simulink model "DWPT_250k_60V_1200W"  (R2026b)
settings: Solver=ode3  StopTime=0.03  FixedStep=Ts  MaxStep=1.0E-7  RelTol=1e-4  AbsTol=1e-6
model workspace (MAT data in the model file):
  CP1 = 8.25994623514e-08
  CS = 4.09933827549e-08
  CT1 = 8.13830913262e-08
  Cout = 0.0022
  Goff = 1e-08
  Ki = 20
  Kp = 0.015
  LP1 = 9.88658918421e-06
  LS = 9.88658918421e-06
  LT1 = 4.97996239716e-06
  M1 = 6.87234810809e-06
  Mdesign = 6.87234810809e-06
  RL = 3
  RP1 = 0.0171021142042
  RS = 0.0171021142042
  RT1 = 0.01
  RonSR = 0.003
  RonTx = 0.003
  Ts = 1e-08
  Vavailable = 69
  Vdc = 50
  Vtarget = 60
  averageCycles = 1250
  bodyRon = 0.01
  bodyVf = 0.8
  closedLoop = 1
  deadTime = 4e-08
  f = 250000
  initialOutputVoltage = 0
  k = 0.695118203056
  samplesPerPeriod = 400
  softStart = 0.02
  srDeadTime = 4e-08
  srEnabled = 1
  srThreshold = 0.25
  voltageHeadroom = 1.15
undefined symbols (not defined in the file or in its folder): ee_sli_rtmsupport, G, gcbh
libraries: sl_signal_attributes x63, eeGeneralControl x37, fl_lib x32, nesl_utility x28, eeGeneralMeasurement x14, ee_lib x8, dspfdesign x1
(part 3 of 3)

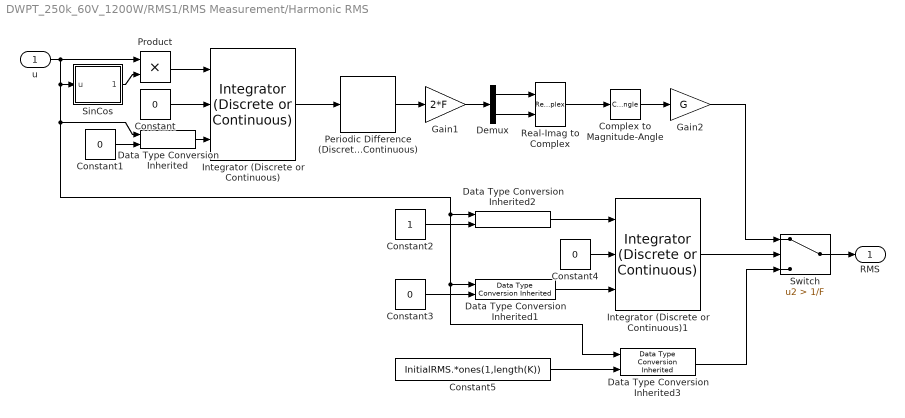
== system DWPT_250k_60V_1200W/RMS1/RMS Measurement/Harmonic RMS ==
  u : Inport
  Complex to Magnitude-Angle : ComplexToMagnitudeAngle  Output=Magnitude
  Constant{,1,3..4} (4 alike) : Constant  Value=0
  Constant2 : Constant
  Constant5 : Constant  Value=InitialRMS.*ones(1,length(K))
  Data Type Conversion Inherited{,1..3} (4 alike) : sl_signal_attributes/Data Type Conversion Inherited  ConvertRealWorld=Real World Value  DoSatur=off
  Demux : Demux  Outputs=2
  Gain1 : Gain  Gain=2*F
  Gain2 : Gain  Gain=G
  Integrator (Discrete or Continuous) : eeGeneralControl/Integrator (Discrete or Continuous)  LabelModeActiveChoice=Continuous  IntegratorMethod=Integration: Forward Euler  ExternalReset=level  LimitType=Anti-windup  B=inf  A=-inf  Ts=Ts
  Integrator (Discrete or Continuous)1 : eeGeneralControl/Integrator (Discrete or Continuous)  LabelModeActiveChoice=Continuous  IntegratorMethod=Integration: Forward Euler  ExternalReset=level  LimitType=Anti-windup  B=2/F  A=-inf  Ts=Ts
  Periodic Difference (Discrete or Continuous) : eeGeneralMeasurement/Periodic Difference (Discrete or Continuous)  LabelModeActiveChoice=Continuous  F=F  Ts=Ts
      link override Continuous/Transport Delay: BufferSize=2^nextpow2(samplesPerPeriod*averageCycles+1024)
  Product : Product
  Real-Imag to Complex : RealImagToComplex
  SinCos : Subsystem
  Switch : Switch  Criteria=u2 > Threshold  Threshold=1/F  SaturateOnIntegerOverflow=off  InputSameDT=off
  RMS : Outport  VectorParamsAs1DForOutWhenUnconnected=off
  wires:
  Switch/1 -> RMS/1
  Gain2/1 -> Switch/1
  Constant2/1 -> Data Type Conversion Inherited2/2
  Constant3/1 -> Data Type Conversion Inherited1/2
  Constant4/1 -> Integrator (Discrete or Continuous)1/2
  Data Type Conversion Inherited3/1 -> Switch/3
  Constant5/1 -> Data Type Conversion Inherited3/2
  Data Type Conversion Inherited2/1 -> Integrator (Discrete or Continuous)1/1
  Data Type Conversion Inherited1/1 -> Integrator (Discrete or Continuous)1/3
  Integrator (Discrete or Continuous)1/1 -> Switch/2
  Constant1/1 -> Data Type Conversion Inherited/2
  Data Type Conversion Inherited/1 -> Integrator (Discrete or Continuous)/3
  Integrator (Discrete or Continuous)/1 -> Periodic Difference (Discrete or Continuous)/1
  Constant/1 -> Integrator (Discrete or Continuous)/2
  Demux/2 -> Real-Imag to Complex/2
  u/1 -> SinCos/1(u), Data Type Conversion Inherited/1, Data Type Conversion Inherited2/1, Data Type Conversion Inherited1/1, Data Type Conversion Inherited3/1, Product/1
  Periodic Difference (Discrete or Continuous)/1 -> Gain1/1
  Real-Imag to Complex/1 -> Complex to Magnitude-Angle/1
  Demux/1 -> Real-Imag to Complex/1
  SinCos/1(SinCos) -> Product/2
  Gain1/1 -> Demux/1
  Product/1 -> Integrator (Discrete or Continuous)/1
  Complex to Magnitude-Angle/1 -> Gain2/1

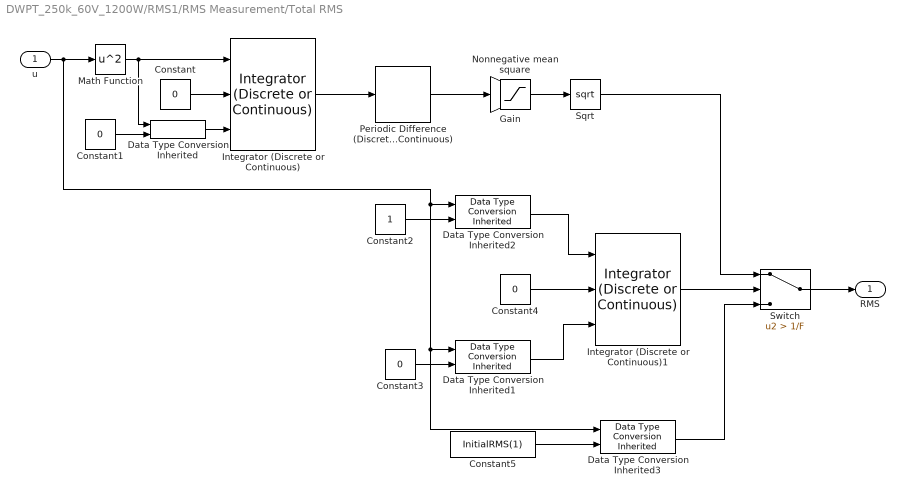
== system DWPT_250k_60V_1200W/RMS1/RMS Measurement/Total RMS ==
  u : Inport
  Constant{,1,3..4} (4 alike) : Constant  Value=0
  Constant2 : Constant
  Constant5 : Constant  Value=InitialRMS(1)
  Data Type Conversion Inherited{,1..3} (4 alike) : sl_signal_attributes/Data Type Conversion Inherited  ConvertRealWorld=Real World Value  DoSatur=off
  Gain : Gain  Gain=F
  Integrator (Discrete or Continuous) : eeGeneralControl/Integrator (Discrete or Continuous)  LabelModeActiveChoice=Continuous  IntegratorMethod=Integration: Forward Euler  ExternalReset=level  LimitType=Anti-windup  B=inf  A=-inf  Ts=Ts
  Integrator (Discrete or Continuous)1 : eeGeneralControl/Integrator (Discrete or Continuous)  LabelModeActiveChoice=Continuous  IntegratorMethod=Integration: Forward Euler  ExternalReset=level  LimitType=Anti-windup  B=2/F  A=-inf  Ts=Ts
  Math Function : Math  Operator=square  SignedPower=on
  Nonnegative mean square : Saturate  UpperLimit=inf  LowerLimit=0
  Periodic Difference (Discrete or Continuous) : eeGeneralMeasurement/Periodic Difference (Discrete or Continuous)  LabelModeActiveChoice=Continuous  F=F  Ts=Ts
      link override Continuous/Transport Delay: BufferSize=2^nextpow2(samplesPerPeriod*averageCycles+1024)
  Sqrt : Sqrt
  Switch : Switch  Criteria=u2 > Threshold  Threshold=1/F  SaturateOnIntegerOverflow=off  InputSameDT=off
  RMS : Outport  VectorParamsAs1DForOutWhenUnconnected=off
  wires:
  Sqrt/1 -> Switch/1
  Switch/1 -> RMS/1
  Constant2/1 -> Data Type Conversion Inherited2/2
  Constant3/1 -> Data Type Conversion Inherited1/2
  Constant4/1 -> Integrator (Discrete or Continuous)1/2
  Data Type Conversion Inherited3/1 -> Switch/3
  Constant5/1 -> Data Type Conversion Inherited3/2
  Data Type Conversion Inherited2/1 -> Integrator (Discrete or Continuous)1/1
  Data Type Conversion Inherited1/1 -> Integrator (Discrete or Continuous)1/3
  Integrator (Discrete or Continuous)1/1 -> Switch/2
  Constant1/1 -> Data Type Conversion Inherited/2
  Data Type Conversion Inherited/1 -> Integrator (Discrete or Continuous)/3
  Periodic Difference (Discrete or Continuous)/1 -> Gain/1
  Integrator (Discrete or Continuous)/1 -> Periodic Difference (Discrete or Continuous)/1
  u/1 -> Math Function/1, Data Type Conversion Inherited2/1, Data Type Conversion Inherited3/1, Data Type Conversion Inherited1/1
  Math Function/1 -> Integrator (Discrete or Continuous)/1, Data Type Conversion Inherited/1
  Constant/1 -> Integrator (Discrete or Continuous)/2
  Gain/1 -> Nonnegative mean square/1
  Nonnegative mean square/1 -> Sqrt/1

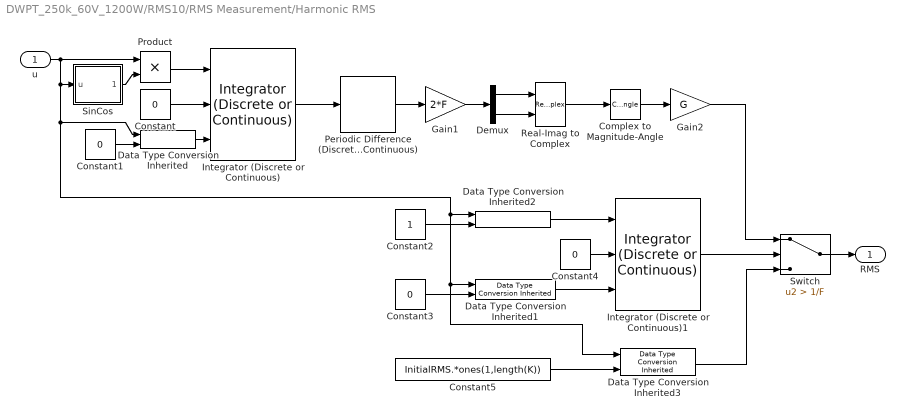
== system DWPT_250k_60V_1200W/RMS10/RMS Measurement/Harmonic RMS ==
  u : Inport
  Complex to Magnitude-Angle : ComplexToMagnitudeAngle  Output=Magnitude
  Constant{,1,3..4} (4 alike) : Constant  Value=0
  Constant2 : Constant
  Constant5 : Constant  Value=InitialRMS.*ones(1,length(K))
  Data Type Conversion Inherited{,1..3} (4 alike) : sl_signal_attributes/Data Type Conversion Inherited  ConvertRealWorld=Real World Value  DoSatur=off
  Demux : Demux  Outputs=2
  Gain1 : Gain  Gain=2*F
  Gain2 : Gain  Gain=G
  Integrator (Discrete or Continuous) : eeGeneralControl/Integrator (Discrete or Continuous)  LabelModeActiveChoice=Continuous  IntegratorMethod=Integration: Forward Euler  ExternalReset=level  LimitType=Anti-windup  B=inf  A=-inf  Ts=Ts
  Integrator (Discrete or Continuous)1 : eeGeneralControl/Integrator (Discrete or Continuous)  LabelModeActiveChoice=Continuous  IntegratorMethod=Integration: Forward Euler  ExternalReset=level  LimitType=Anti-windup  B=2/F  A=-inf  Ts=Ts
  Periodic Difference (Discrete or Continuous) : eeGeneralMeasurement/Periodic Difference (Discrete or Continuous)  LabelModeActiveChoice=Continuous  F=F  Ts=Ts
      link override Continuous/Transport Delay: BufferSize=2^nextpow2(samplesPerPeriod*averageCycles+1024)
  Product : Product
  Real-Imag to Complex : RealImagToComplex
  SinCos : Subsystem
  Switch : Switch  Criteria=u2 > Threshold  Threshold=1/F  SaturateOnIntegerOverflow=off  InputSameDT=off
  RMS : Outport  VectorParamsAs1DForOutWhenUnconnected=off
  wires:
  Switch/1 -> RMS/1
  Gain2/1 -> Switch/1
  Constant2/1 -> Data Type Conversion Inherited2/2
  Constant3/1 -> Data Type Conversion Inherited1/2
  Constant4/1 -> Integrator (Discrete or Continuous)1/2
  Data Type Conversion Inherited3/1 -> Switch/3
  Constant5/1 -> Data Type Conversion Inherited3/2
  Data Type Conversion Inherited2/1 -> Integrator (Discrete or Continuous)1/1
  Data Type Conversion Inherited1/1 -> Integrator (Discrete or Continuous)1/3
  Integrator (Discrete or Continuous)1/1 -> Switch/2
  Constant1/1 -> Data Type Conversion Inherited/2
  Data Type Conversion Inherited/1 -> Integrator (Discrete or Continuous)/3
  Integrator (Discrete or Continuous)/1 -> Periodic Difference (Discrete or Continuous)/1
  Constant/1 -> Integrator (Discrete or Continuous)/2
  Demux/2 -> Real-Imag to Complex/2
  u/1 -> SinCos/1(u), Data Type Conversion Inherited/1, Data Type Conversion Inherited2/1, Data Type Conversion Inherited1/1, Data Type Conversion Inherited3/1, Product/1
  Periodic Difference (Discrete or Continuous)/1 -> Gain1/1
  Real-Imag to Complex/1 -> Complex to Magnitude-Angle/1
  Demux/1 -> Real-Imag to Complex/1
  SinCos/1(SinCos) -> Product/2
  Gain1/1 -> Demux/1
  Product/1 -> Integrator (Discrete or Continuous)/1
  Complex to Magnitude-Angle/1 -> Gain2/1

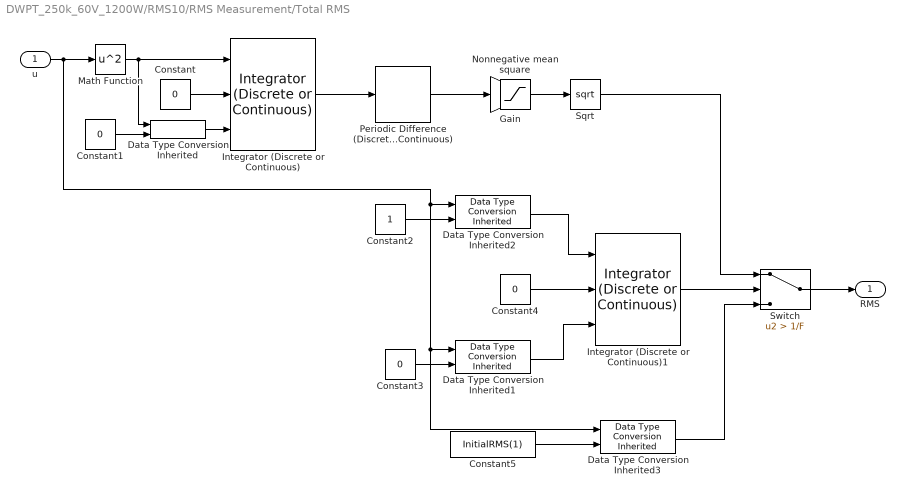
== system DWPT_250k_60V_1200W/RMS10/RMS Measurement/Total RMS ==
  u : Inport
  Constant{,1,3..4} (4 alike) : Constant  Value=0
  Constant2 : Constant
  Constant5 : Constant  Value=InitialRMS(1)
  Data Type Conversion Inherited{,1..3} (4 alike) : sl_signal_attributes/Data Type Conversion Inherited  ConvertRealWorld=Real World Value  DoSatur=off
  Gain : Gain  Gain=F
  Integrator (Discrete or Continuous) : eeGeneralControl/Integrator (Discrete or Continuous)  LabelModeActiveChoice=Continuous  IntegratorMethod=Integration: Forward Euler  ExternalReset=level  LimitType=Anti-windup  B=inf  A=-inf  Ts=Ts
  Integrator (Discrete or Continuous)1 : eeGeneralControl/Integrator (Discrete or Continuous)  LabelModeActiveChoice=Continuous  IntegratorMethod=Integration: Forward Euler  ExternalReset=level  LimitType=Anti-windup  B=2/F  A=-inf  Ts=Ts
  Math Function : Math  Operator=square  SignedPower=on
  Nonnegative mean square : Saturate  UpperLimit=inf  LowerLimit=0
  Periodic Difference (Discrete or Continuous) : eeGeneralMeasurement/Periodic Difference (Discrete or Continuous)  LabelModeActiveChoice=Continuous  F=F  Ts=Ts
      link override Continuous/Transport Delay: BufferSize=2^nextpow2(samplesPerPeriod*averageCycles+1024)
  Sqrt : Sqrt
  Switch : Switch  Criteria=u2 > Threshold  Threshold=1/F  SaturateOnIntegerOverflow=off  InputSameDT=off
  RMS : Outport  VectorParamsAs1DForOutWhenUnconnected=off
  wires:
  Sqrt/1 -> Switch/1
  Switch/1 -> RMS/1
  Constant2/1 -> Data Type Conversion Inherited2/2
  Constant3/1 -> Data Type Conversion Inherited1/2
  Constant4/1 -> Integrator (Discrete or Continuous)1/2
  Data Type Conversion Inherited3/1 -> Switch/3
  Constant5/1 -> Data Type Conversion Inherited3/2
  Data Type Conversion Inherited2/1 -> Integrator (Discrete or Continuous)1/1
  Data Type Conversion Inherited1/1 -> Integrator (Discrete or Continuous)1/3
  Integrator (Discrete or Continuous)1/1 -> Switch/2
  Constant1/1 -> Data Type Conversion Inherited/2
  Data Type Conversion Inherited/1 -> Integrator (Discrete or Continuous)/3
  Periodic Difference (Discrete or Continuous)/1 -> Gain/1
  Integrator (Discrete or Continuous)/1 -> Periodic Difference (Discrete or Continuous)/1
  u/1 -> Math Function/1, Data Type Conversion Inherited2/1, Data Type Conversion Inherited3/1, Data Type Conversion Inherited1/1
  Math Function/1 -> Integrator (Discrete or Continuous)/1, Data Type Conversion Inherited/1
  Constant/1 -> Integrator (Discrete or Continuous)/2
  Gain/1 -> Nonnegative mean square/1
  Nonnegative mean square/1 -> Sqrt/1

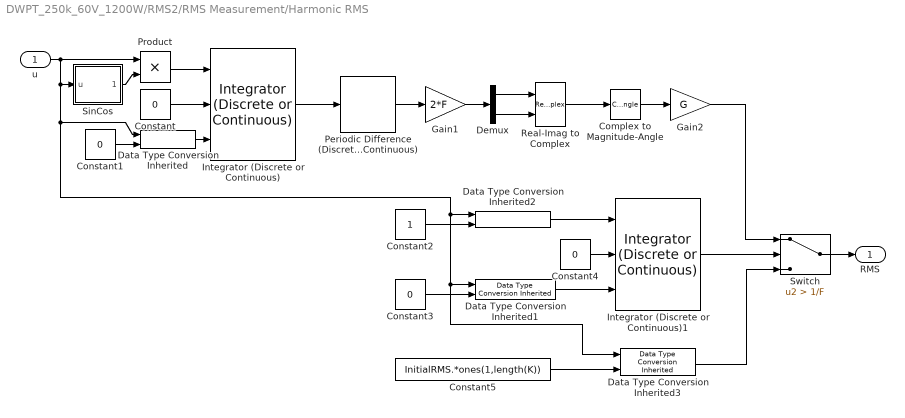
== system DWPT_250k_60V_1200W/RMS2/RMS Measurement/Harmonic RMS ==
  u : Inport
  Complex to Magnitude-Angle : ComplexToMagnitudeAngle  Output=Magnitude
  Constant{,1,3..4} (4 alike) : Constant  Value=0
  Constant2 : Constant
  Constant5 : Constant  Value=InitialRMS.*ones(1,length(K))
  Data Type Conversion Inherited{,1..3} (4 alike) : sl_signal_attributes/Data Type Conversion Inherited  ConvertRealWorld=Real World Value  DoSatur=off
  Demux : Demux  Outputs=2
  Gain1 : Gain  Gain=2*F
  Gain2 : Gain  Gain=G
  Integrator (Discrete or Continuous) : eeGeneralControl/Integrator (Discrete or Continuous)  LabelModeActiveChoice=Continuous  IntegratorMethod=Integration: Forward Euler  ExternalReset=level  LimitType=Anti-windup  B=inf  A=-inf  Ts=Ts
  Integrator (Discrete or Continuous)1 : eeGeneralControl/Integrator (Discrete or Continuous)  LabelModeActiveChoice=Continuous  IntegratorMethod=Integration: Forward Euler  ExternalReset=level  LimitType=Anti-windup  B=2/F  A=-inf  Ts=Ts
  Periodic Difference (Discrete or Continuous) : eeGeneralMeasurement/Periodic Difference (Discrete or Continuous)  LabelModeActiveChoice=Continuous  F=F  Ts=Ts
      link override Continuous/Transport Delay: BufferSize=2^nextpow2(samplesPerPeriod*averageCycles+1024)
  Product : Product
  Real-Imag to Complex : RealImagToComplex
  SinCos : Subsystem
  Switch : Switch  Criteria=u2 > Threshold  Threshold=1/F  SaturateOnIntegerOverflow=off  InputSameDT=off
  RMS : Outport  VectorParamsAs1DForOutWhenUnconnected=off
  wires:
  Switch/1 -> RMS/1
  Gain2/1 -> Switch/1
  Constant2/1 -> Data Type Conversion Inherited2/2
  Constant3/1 -> Data Type Conversion Inherited1/2
  Constant4/1 -> Integrator (Discrete or Continuous)1/2
  Data Type Conversion Inherited3/1 -> Switch/3
  Constant5/1 -> Data Type Conversion Inherited3/2
  Data Type Conversion Inherited2/1 -> Integrator (Discrete or Continuous)1/1
  Data Type Conversion Inherited1/1 -> Integrator (Discrete or Continuous)1/3
  Integrator (Discrete or Continuous)1/1 -> Switch/2
  Constant1/1 -> Data Type Conversion Inherited/2
  Data Type Conversion Inherited/1 -> Integrator (Discrete or Continuous)/3
  Integrator (Discrete or Continuous)/1 -> Periodic Difference (Discrete or Continuous)/1
  Constant/1 -> Integrator (Discrete or Continuous)/2
  Demux/2 -> Real-Imag to Complex/2
  u/1 -> SinCos/1(u), Data Type Conversion Inherited/1, Data Type Conversion Inherited2/1, Data Type Conversion Inherited1/1, Data Type Conversion Inherited3/1, Product/1
  Periodic Difference (Discrete or Continuous)/1 -> Gain1/1
  Real-Imag to Complex/1 -> Complex to Magnitude-Angle/1
  Demux/1 -> Real-Imag to Complex/1
  SinCos/1(SinCos) -> Product/2
  Gain1/1 -> Demux/1
  Product/1 -> Integrator (Discrete or Continuous)/1
  Complex to Magnitude-Angle/1 -> Gain2/1

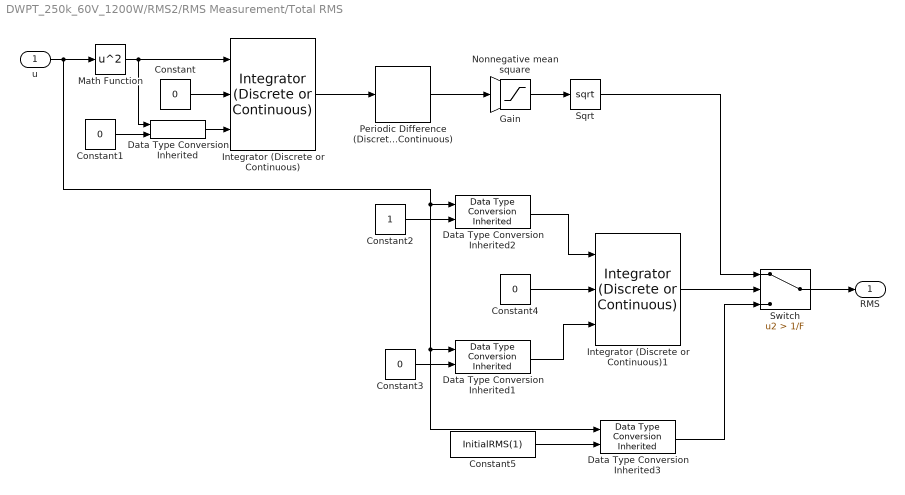
== system DWPT_250k_60V_1200W/RMS2/RMS Measurement/Total RMS ==
  u : Inport
  Constant{,1,3..4} (4 alike) : Constant  Value=0
  Constant2 : Constant
  Constant5 : Constant  Value=InitialRMS(1)
  Data Type Conversion Inherited{,1..3} (4 alike) : sl_signal_attributes/Data Type Conversion Inherited  ConvertRealWorld=Real World Value  DoSatur=off
  Gain : Gain  Gain=F
  Integrator (Discrete or Continuous) : eeGeneralControl/Integrator (Discrete or Continuous)  LabelModeActiveChoice=Continuous  IntegratorMethod=Integration: Forward Euler  ExternalReset=level  LimitType=Anti-windup  B=inf  A=-inf  Ts=Ts
  Integrator (Discrete or Continuous)1 : eeGeneralControl/Integrator (Discrete or Continuous)  LabelModeActiveChoice=Continuous  IntegratorMethod=Integration: Forward Euler  ExternalReset=level  LimitType=Anti-windup  B=2/F  A=-inf  Ts=Ts
  Math Function : Math  Operator=square  SignedPower=on
  Nonnegative mean square : Saturate  UpperLimit=inf  LowerLimit=0
  Periodic Difference (Discrete or Continuous) : eeGeneralMeasurement/Periodic Difference (Discrete or Continuous)  LabelModeActiveChoice=Continuous  F=F  Ts=Ts
      link override Continuous/Transport Delay: BufferSize=2^nextpow2(samplesPerPeriod*averageCycles+1024)
  Sqrt : Sqrt
  Switch : Switch  Criteria=u2 > Threshold  Threshold=1/F  SaturateOnIntegerOverflow=off  InputSameDT=off
  RMS : Outport  VectorParamsAs1DForOutWhenUnconnected=off
  wires:
  Sqrt/1 -> Switch/1
  Switch/1 -> RMS/1
  Constant2/1 -> Data Type Conversion Inherited2/2
  Constant3/1 -> Data Type Conversion Inherited1/2
  Constant4/1 -> Integrator (Discrete or Continuous)1/2
  Data Type Conversion Inherited3/1 -> Switch/3
  Constant5/1 -> Data Type Conversion Inherited3/2
  Data Type Conversion Inherited2/1 -> Integrator (Discrete or Continuous)1/1
  Data Type Conversion Inherited1/1 -> Integrator (Discrete or Continuous)1/3
  Integrator (Discrete or Continuous)1/1 -> Switch/2
  Constant1/1 -> Data Type Conversion Inherited/2
  Data Type Conversion Inherited/1 -> Integrator (Discrete or Continuous)/3
  Periodic Difference (Discrete or Continuous)/1 -> Gain/1
  Integrator (Discrete or Continuous)/1 -> Periodic Difference (Discrete or Continuous)/1
  u/1 -> Math Function/1, Data Type Conversion Inherited2/1, Data Type Conversion Inherited3/1, Data Type Conversion Inherited1/1
  Math Function/1 -> Integrator (Discrete or Continuous)/1, Data Type Conversion Inherited/1
  Constant/1 -> Integrator (Discrete or Continuous)/2
  Gain/1 -> Nonnegative mean square/1
  Nonnegative mean square/1 -> Sqrt/1

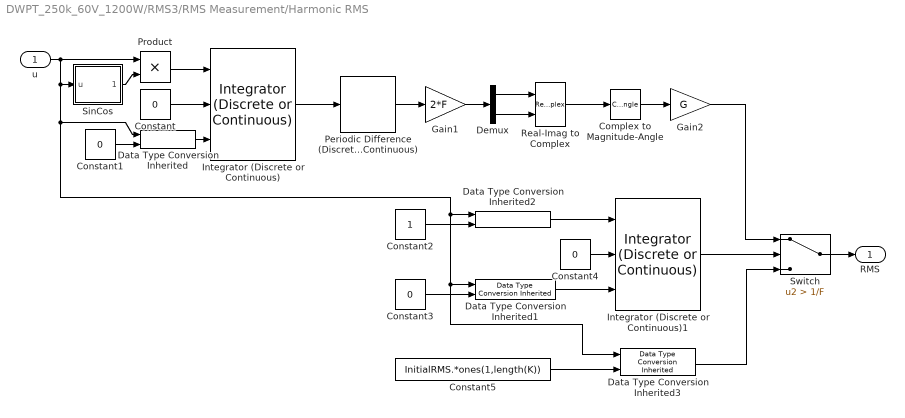
== system DWPT_250k_60V_1200W/RMS3/RMS Measurement/Harmonic RMS ==
  u : Inport
  Complex to Magnitude-Angle : ComplexToMagnitudeAngle  Output=Magnitude
  Constant{,1,3..4} (4 alike) : Constant  Value=0
  Constant2 : Constant
  Constant5 : Constant  Value=InitialRMS.*ones(1,length(K))
  Data Type Conversion Inherited{,1..3} (4 alike) : sl_signal_attributes/Data Type Conversion Inherited  ConvertRealWorld=Real World Value  DoSatur=off
  Demux : Demux  Outputs=2
  Gain1 : Gain  Gain=2*F
  Gain2 : Gain  Gain=G
  Integrator (Discrete or Continuous) : eeGeneralControl/Integrator (Discrete or Continuous)  LabelModeActiveChoice=Continuous  IntegratorMethod=Integration: Forward Euler  ExternalReset=level  LimitType=Anti-windup  B=inf  A=-inf  Ts=Ts
  Integrator (Discrete or Continuous)1 : eeGeneralControl/Integrator (Discrete or Continuous)  LabelModeActiveChoice=Continuous  IntegratorMethod=Integration: Forward Euler  ExternalReset=level  LimitType=Anti-windup  B=2/F  A=-inf  Ts=Ts
  Periodic Difference (Discrete or Continuous) : eeGeneralMeasurement/Periodic Difference (Discrete or Continuous)  LabelModeActiveChoice=Continuous  F=F  Ts=Ts
      link override Continuous/Transport Delay: BufferSize=2^nextpow2(samplesPerPeriod*averageCycles+1024)
  Product : Product
  Real-Imag to Complex : RealImagToComplex
  SinCos : Subsystem
  Switch : Switch  Criteria=u2 > Threshold  Threshold=1/F  SaturateOnIntegerOverflow=off  InputSameDT=off
  RMS : Outport  VectorParamsAs1DForOutWhenUnconnected=off
  wires:
  Switch/1 -> RMS/1
  Gain2/1 -> Switch/1
  Constant2/1 -> Data Type Conversion Inherited2/2
  Constant3/1 -> Data Type Conversion Inherited1/2
  Constant4/1 -> Integrator (Discrete or Continuous)1/2
  Data Type Conversion Inherited3/1 -> Switch/3
  Constant5/1 -> Data Type Conversion Inherited3/2
  Data Type Conversion Inherited2/1 -> Integrator (Discrete or Continuous)1/1
  Data Type Conversion Inherited1/1 -> Integrator (Discrete or Continuous)1/3
  Integrator (Discrete or Continuous)1/1 -> Switch/2
  Constant1/1 -> Data Type Conversion Inherited/2
  Data Type Conversion Inherited/1 -> Integrator (Discrete or Continuous)/3
  Integrator (Discrete or Continuous)/1 -> Periodic Difference (Discrete or Continuous)/1
  Constant/1 -> Integrator (Discrete or Continuous)/2
  Demux/2 -> Real-Imag to Complex/2
  u/1 -> SinCos/1(u), Data Type Conversion Inherited/1, Data Type Conversion Inherited2/1, Data Type Conversion Inherited1/1, Data Type Conversion Inherited3/1, Product/1
  Periodic Difference (Discrete or Continuous)/1 -> Gain1/1
  Real-Imag to Complex/1 -> Complex to Magnitude-Angle/1
  Demux/1 -> Real-Imag to Complex/1
  SinCos/1(SinCos) -> Product/2
  Gain1/1 -> Demux/1
  Product/1 -> Integrator (Discrete or Continuous)/1
  Complex to Magnitude-Angle/1 -> Gain2/1

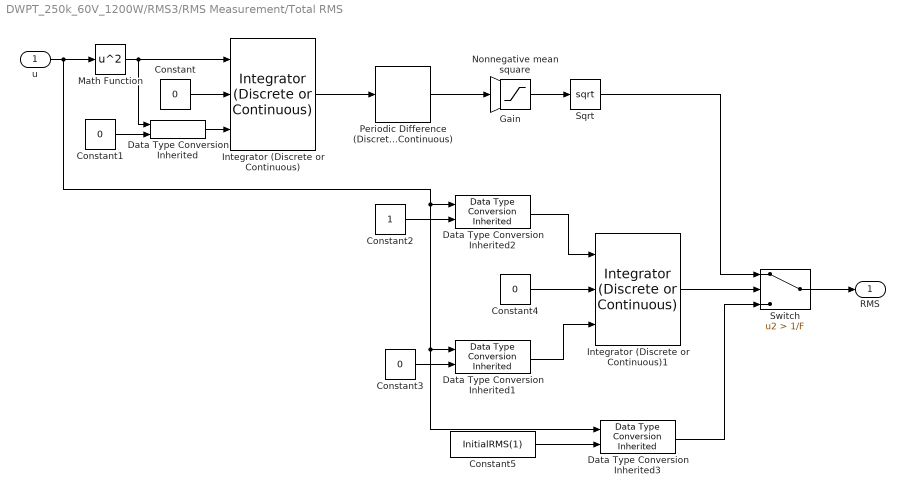
== system DWPT_250k_60V_1200W/RMS3/RMS Measurement/Total RMS ==
  u : Inport
  Constant{,1,3..4} (4 alike) : Constant  Value=0
  Constant2 : Constant
  Constant5 : Constant  Value=InitialRMS(1)
  Data Type Conversion Inherited{,1..3} (4 alike) : sl_signal_attributes/Data Type Conversion Inherited  ConvertRealWorld=Real World Value  DoSatur=off
  Gain : Gain  Gain=F
  Integrator (Discrete or Continuous) : eeGeneralControl/Integrator (Discrete or Continuous)  LabelModeActiveChoice=Continuous  IntegratorMethod=Integration: Forward Euler  ExternalReset=level  LimitType=Anti-windup  B=inf  A=-inf  Ts=Ts
  Integrator (Discrete or Continuous)1 : eeGeneralControl/Integrator (Discrete or Continuous)  LabelModeActiveChoice=Continuous  IntegratorMethod=Integration: Forward Euler  ExternalReset=level  LimitType=Anti-windup  B=2/F  A=-inf  Ts=Ts
  Math Function : Math  Operator=square  SignedPower=on
  Nonnegative mean square : Saturate  UpperLimit=inf  LowerLimit=0
  Periodic Difference (Discrete or Continuous) : eeGeneralMeasurement/Periodic Difference (Discrete or Continuous)  LabelModeActiveChoice=Continuous  F=F  Ts=Ts
      link override Continuous/Transport Delay: BufferSize=2^nextpow2(samplesPerPeriod*averageCycles+1024)
  Sqrt : Sqrt
  Switch : Switch  Criteria=u2 > Threshold  Threshold=1/F  SaturateOnIntegerOverflow=off  InputSameDT=off
  RMS : Outport  VectorParamsAs1DForOutWhenUnconnected=off
  wires:
  Sqrt/1 -> Switch/1
  Switch/1 -> RMS/1
  Constant2/1 -> Data Type Conversion Inherited2/2
  Constant3/1 -> Data Type Conversion Inherited1/2
  Constant4/1 -> Integrator (Discrete or Continuous)1/2
  Data Type Conversion Inherited3/1 -> Switch/3
  Constant5/1 -> Data Type Conversion Inherited3/2
  Data Type Conversion Inherited2/1 -> Integrator (Discrete or Continuous)1/1
  Data Type Conversion Inherited1/1 -> Integrator (Discrete or Continuous)1/3
  Integrator (Discrete or Continuous)1/1 -> Switch/2
  Constant1/1 -> Data Type Conversion Inherited/2
  Data Type Conversion Inherited/1 -> Integrator (Discrete or Continuous)/3
  Periodic Difference (Discrete or Continuous)/1 -> Gain/1
  Integrator (Discrete or Continuous)/1 -> Periodic Difference (Discrete or Continuous)/1
  u/1 -> Math Function/1, Data Type Conversion Inherited2/1, Data Type Conversion Inherited3/1, Data Type Conversion Inherited1/1
  Math Function/1 -> Integrator (Discrete or Continuous)/1, Data Type Conversion Inherited/1
  Constant/1 -> Integrator (Discrete or Continuous)/2
  Gain/1 -> Nonnegative mean square/1
  Nonnegative mean square/1 -> Sqrt/1

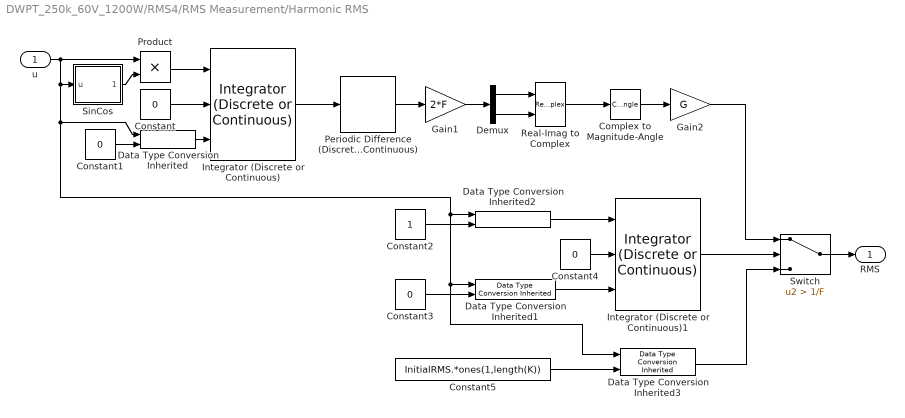
== system DWPT_250k_60V_1200W/RMS4/RMS Measurement/Harmonic RMS ==
  u : Inport
  Complex to Magnitude-Angle : ComplexToMagnitudeAngle  Output=Magnitude
  Constant{,1,3..4} (4 alike) : Constant  Value=0
  Constant2 : Constant
  Constant5 : Constant  Value=InitialRMS.*ones(1,length(K))
  Data Type Conversion Inherited{,1..3} (4 alike) : sl_signal_attributes/Data Type Conversion Inherited  ConvertRealWorld=Real World Value  DoSatur=off
  Demux : Demux  Outputs=2
  Gain1 : Gain  Gain=2*F
  Gain2 : Gain  Gain=G
  Integrator (Discrete or Continuous) : eeGeneralControl/Integrator (Discrete or Continuous)  LabelModeActiveChoice=Continuous  IntegratorMethod=Integration: Forward Euler  ExternalReset=level  LimitType=Anti-windup  B=inf  A=-inf  Ts=Ts
  Integrator (Discrete or Continuous)1 : eeGeneralControl/Integrator (Discrete or Continuous)  LabelModeActiveChoice=Continuous  IntegratorMethod=Integration: Forward Euler  ExternalReset=level  LimitType=Anti-windup  B=2/F  A=-inf  Ts=Ts
  Periodic Difference (Discrete or Continuous) : eeGeneralMeasurement/Periodic Difference (Discrete or Continuous)  LabelModeActiveChoice=Continuous  F=F  Ts=Ts
      link override Continuous/Transport Delay: BufferSize=2^nextpow2(samplesPerPeriod*averageCycles+1024)
  Product : Product
  Real-Imag to Complex : RealImagToComplex
  SinCos : Subsystem
  Switch : Switch  Criteria=u2 > Threshold  Threshold=1/F  SaturateOnIntegerOverflow=off  InputSameDT=off
  RMS : Outport  VectorParamsAs1DForOutWhenUnconnected=off
  wires:
  Switch/1 -> RMS/1
  Gain2/1 -> Switch/1
  Constant2/1 -> Data Type Conversion Inherited2/2
  Constant3/1 -> Data Type Conversion Inherited1/2
  Constant4/1 -> Integrator (Discrete or Continuous)1/2
  Data Type Conversion Inherited3/1 -> Switch/3
  Constant5/1 -> Data Type Conversion Inherited3/2
  Data Type Conversion Inherited2/1 -> Integrator (Discrete or Continuous)1/1
  Data Type Conversion Inherited1/1 -> Integrator (Discrete or Continuous)1/3
  Integrator (Discrete or Continuous)1/1 -> Switch/2
  Constant1/1 -> Data Type Conversion Inherited/2
  Data Type Conversion Inherited/1 -> Integrator (Discrete or Continuous)/3
  Integrator (Discrete or Continuous)/1 -> Periodic Difference (Discrete or Continuous)/1
  Constant/1 -> Integrator (Discrete or Continuous)/2
  Demux/2 -> Real-Imag to Complex/2
  u/1 -> SinCos/1(u), Data Type Conversion Inherited/1, Data Type Conversion Inherited2/1, Data Type Conversion Inherited1/1, Data Type Conversion Inherited3/1, Product/1
  Periodic Difference (Discrete or Continuous)/1 -> Gain1/1
  Real-Imag to Complex/1 -> Complex to Magnitude-Angle/1
  Demux/1 -> Real-Imag to Complex/1
  SinCos/1(SinCos) -> Product/2
  Gain1/1 -> Demux/1
  Product/1 -> Integrator (Discrete or Continuous)/1
  Complex to Magnitude-Angle/1 -> Gain2/1

== system DWPT_250k_60V_1200W/RMS4/RMS Measurement/Total RMS ==
  u : Inport
  Constant{,1,3..4} (4 alike) : Constant  Value=0
  Constant2 : Constant
  Constant5 : Constant  Value=InitialRMS(1)
  Data Type Conversion Inherited{,1..3} (4 alike) : sl_signal_attributes/Data Type Conversion Inherited  ConvertRealWorld=Real World Value  DoSatur=off
  Gain : Gain  Gain=F
  Integrator (Discrete or Continuous) : eeGeneralControl/Integrator (Discrete or Continuous)  LabelModeActiveChoice=Continuous  IntegratorMethod=Integration: Forward Euler  ExternalReset=level  LimitType=Anti-windup  B=inf  A=-inf  Ts=Ts
  Integrator (Discrete or Continuous)1 : eeGeneralControl/Integrator (Discrete or Continuous)  LabelModeActiveChoice=Continuous  IntegratorMethod=Integration: Forward Euler  ExternalReset=level  LimitType=Anti-windup  B=2/F  A=-inf  Ts=Ts
  Math Function : Math  Operator=square  SignedPower=on
  Nonnegative mean square : Saturate  UpperLimit=inf  LowerLimit=0
  Periodic Difference (Discrete or Continuous) : eeGeneralMeasurement/Periodic Difference (Discrete or Continuous)  LabelModeActiveChoice=Continuous  F=F  Ts=Ts
      link override Continuous/Transport Delay: BufferSize=2^nextpow2(samplesPerPeriod*averageCycles+1024)
  Sqrt : Sqrt
  Switch : Switch  Criteria=u2 > Threshold  Threshold=1/F  SaturateOnIntegerOverflow=off  InputSameDT=off
  RMS : Outport  VectorParamsAs1DForOutWhenUnconnected=off
  wires:
  Sqrt/1 -> Switch/1
  Switch/1 -> RMS/1
  Constant2/1 -> Data Type Conversion Inherited2/2
  Constant3/1 -> Data Type Conversion Inherited1/2
  Constant4/1 -> Integrator (Discrete or Continuous)1/2
  Data Type Conversion Inherited3/1 -> Switch/3
  Constant5/1 -> Data Type Conversion Inherited3/2
  Data Type Conversion Inherited2/1 -> Integrator (Discrete or Continuous)1/1
  Data Type Conversion Inherited1/1 -> Integrator (Discrete or Continuous)1/3
  Integrator (Discrete or Continuous)1/1 -> Switch/2
  Constant1/1 -> Data Type Conversion Inherited/2
  Data Type Conversion Inherited/1 -> Integrator (Discrete or Continuous)/3
  Periodic Difference (Discrete or Continuous)/1 -> Gain/1
  Integrator (Discrete or Continuous)/1 -> Periodic Difference (Discrete or Continuous)/1
  u/1 -> Math Function/1, Data Type Conversion Inherited2/1, Data Type Conversion Inherited3/1, Data Type Conversion Inherited1/1
  Math Function/1 -> Integrator (Discrete or Continuous)/1, Data Type Conversion Inherited/1
  Constant/1 -> Integrator (Discrete or Continuous)/2
  Gain/1 -> Nonnegative mean square/1
  Nonnegative mean square/1 -> Sqrt/1

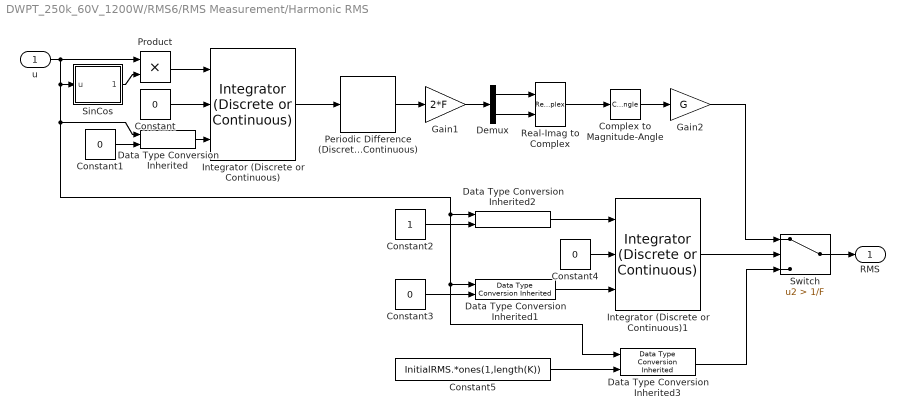
== system DWPT_250k_60V_1200W/RMS6/RMS Measurement/Harmonic RMS ==
  u : Inport
  Complex to Magnitude-Angle : ComplexToMagnitudeAngle  Output=Magnitude
  Constant{,1,3..4} (4 alike) : Constant  Value=0
  Constant2 : Constant
  Constant5 : Constant  Value=InitialRMS.*ones(1,length(K))
  Data Type Conversion Inherited{,1..3} (4 alike) : sl_signal_attributes/Data Type Conversion Inherited  ConvertRealWorld=Real World Value  DoSatur=off
  Demux : Demux  Outputs=2
  Gain1 : Gain  Gain=2*F
  Gain2 : Gain  Gain=G
  Integrator (Discrete or Continuous) : eeGeneralControl/Integrator (Discrete or Continuous)  LabelModeActiveChoice=Continuous  IntegratorMethod=Integration: Forward Euler  ExternalReset=level  LimitType=Anti-windup  B=inf  A=-inf  Ts=Ts
  Integrator (Discrete or Continuous)1 : eeGeneralControl/Integrator (Discrete or Continuous)  LabelModeActiveChoice=Continuous  IntegratorMethod=Integration: Forward Euler  ExternalReset=level  LimitType=Anti-windup  B=2/F  A=-inf  Ts=Ts
  Periodic Difference (Discrete or Continuous) : eeGeneralMeasurement/Periodic Difference (Discrete or Continuous)  LabelModeActiveChoice=Continuous  F=F  Ts=Ts
      link override Continuous/Transport Delay: BufferSize=2^nextpow2(samplesPerPeriod*averageCycles+1024)
  Product : Product
  Real-Imag to Complex : RealImagToComplex
  SinCos : Subsystem
  Switch : Switch  Criteria=u2 > Threshold  Threshold=1/F  SaturateOnIntegerOverflow=off  InputSameDT=off
  RMS : Outport  VectorParamsAs1DForOutWhenUnconnected=off
  wires:
  Switch/1 -> RMS/1
  Gain2/1 -> Switch/1
  Constant2/1 -> Data Type Conversion Inherited2/2
  Constant3/1 -> Data Type Conversion Inherited1/2
  Constant4/1 -> Integrator (Discrete or Continuous)1/2
  Data Type Conversion Inherited3/1 -> Switch/3
  Constant5/1 -> Data Type Conversion Inherited3/2
  Data Type Conversion Inherited2/1 -> Integrator (Discrete or Continuous)1/1
  Data Type Conversion Inherited1/1 -> Integrator (Discrete or Continuous)1/3
  Integrator (Discrete or Continuous)1/1 -> Switch/2
  Constant1/1 -> Data Type Conversion Inherited/2
  Data Type Conversion Inherited/1 -> Integrator (Discrete or Continuous)/3
  Integrator (Discrete or Continuous)/1 -> Periodic Difference (Discrete or Continuous)/1
  Constant/1 -> Integrator (Discrete or Continuous)/2
  Demux/2 -> Real-Imag to Complex/2
  u/1 -> SinCos/1(u), Data Type Conversion Inherited/1, Data Type Conversion Inherited2/1, Data Type Conversion Inherited1/1, Data Type Conversion Inherited3/1, Product/1
  Periodic Difference (Discrete or Continuous)/1 -> Gain1/1
  Real-Imag to Complex/1 -> Complex to Magnitude-Angle/1
  Demux/1 -> Real-Imag to Complex/1
  SinCos/1(SinCos) -> Product/2
  Gain1/1 -> Demux/1
  Product/1 -> Integrator (Discrete or Continuous)/1
  Complex to Magnitude-Angle/1 -> Gain2/1

== system DWPT_250k_60V_1200W/RMS6/RMS Measurement/Total RMS ==
  u : Inport
  Constant{,1,3..4} (4 alike) : Constant  Value=0
  Constant2 : Constant
  Constant5 : Constant  Value=InitialRMS(1)
  Data Type Conversion Inherited{,1..3} (4 alike) : sl_signal_attributes/Data Type Conversion Inherited  ConvertRealWorld=Real World Value  DoSatur=off
  Gain : Gain  Gain=F
  Integrator (Discrete or Continuous) : eeGeneralControl/Integrator (Discrete or Continuous)  LabelModeActiveChoice=Continuous  IntegratorMethod=Integration: Forward Euler  ExternalReset=level  LimitType=Anti-windup  B=inf  A=-inf  Ts=Ts
  Integrator (Discrete or Continuous)1 : eeGeneralControl/Integrator (Discrete or Continuous)  LabelModeActiveChoice=Continuous  IntegratorMethod=Integration: Forward Euler  ExternalReset=level  LimitType=Anti-windup  B=2/F  A=-inf  Ts=Ts
  Math Function : Math  Operator=square  SignedPower=on
  Nonnegative mean square : Saturate  UpperLimit=inf  LowerLimit=0
  Periodic Difference (Discrete or Continuous) : eeGeneralMeasurement/Periodic Difference (Discrete or Continuous)  LabelModeActiveChoice=Continuous  F=F  Ts=Ts
      link override Continuous/Transport Delay: BufferSize=2^nextpow2(samplesPerPeriod*averageCycles+1024)
  Sqrt : Sqrt
  Switch : Switch  Criteria=u2 > Threshold  Threshold=1/F  SaturateOnIntegerOverflow=off  InputSameDT=off
  RMS : Outport  VectorParamsAs1DForOutWhenUnconnected=off
  wires:
  Sqrt/1 -> Switch/1
  Switch/1 -> RMS/1
  Constant2/1 -> Data Type Conversion Inherited2/2
  Constant3/1 -> Data Type Conversion Inherited1/2
  Constant4/1 -> Integrator (Discrete or Continuous)1/2
  Data Type Conversion Inherited3/1 -> Switch/3
  Constant5/1 -> Data Type Conversion Inherited3/2
  Data Type Conversion Inherited2/1 -> Integrator (Discrete or Continuous)1/1
  Data Type Conversion Inherited1/1 -> Integrator (Discrete or Continuous)1/3
  Integrator (Discrete or Continuous)1/1 -> Switch/2
  Constant1/1 -> Data Type Conversion Inherited/2
  Data Type Conversion Inherited/1 -> Integrator (Discrete or Continuous)/3
  Periodic Difference (Discrete or Continuous)/1 -> Gain/1
  Integrator (Discrete or Continuous)/1 -> Periodic Difference (Discrete or Continuous)/1
  u/1 -> Math Function/1, Data Type Conversion Inherited2/1, Data Type Conversion Inherited3/1, Data Type Conversion Inherited1/1
  Math Function/1 -> Integrator (Discrete or Continuous)/1, Data Type Conversion Inherited/1
  Constant/1 -> Integrator (Discrete or Continuous)/2
  Gain/1 -> Nonnegative mean square/1
  Nonnegative mean square/1 -> Sqrt/1

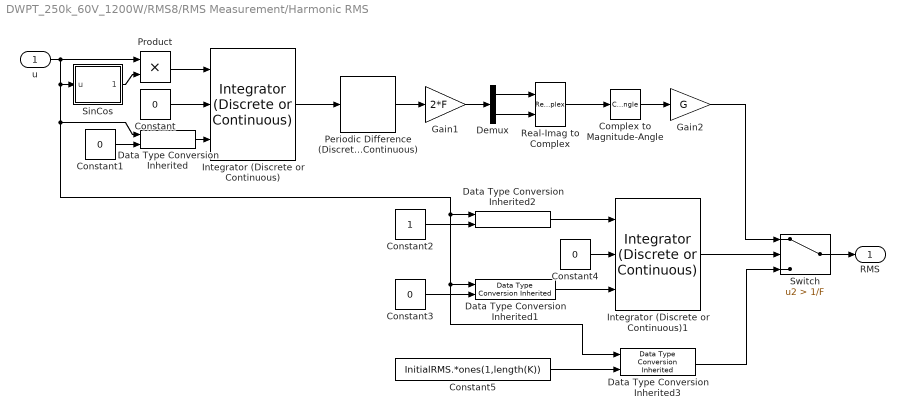
== system DWPT_250k_60V_1200W/RMS8/RMS Measurement/Harmonic RMS ==
  u : Inport
  Complex to Magnitude-Angle : ComplexToMagnitudeAngle  Output=Magnitude
  Constant{,1,3..4} (4 alike) : Constant  Value=0
  Constant2 : Constant
  Constant5 : Constant  Value=InitialRMS.*ones(1,length(K))
  Data Type Conversion Inherited{,1..3} (4 alike) : sl_signal_attributes/Data Type Conversion Inherited  ConvertRealWorld=Real World Value  DoSatur=off
  Demux : Demux  Outputs=2
  Gain1 : Gain  Gain=2*F
  Gain2 : Gain  Gain=G
  Integrator (Discrete or Continuous) : eeGeneralControl/Integrator (Discrete or Continuous)  LabelModeActiveChoice=Continuous  IntegratorMethod=Integration: Forward Euler  ExternalReset=level  LimitType=Anti-windup  B=inf  A=-inf  Ts=Ts
  Integrator (Discrete or Continuous)1 : eeGeneralControl/Integrator (Discrete or Continuous)  LabelModeActiveChoice=Continuous  IntegratorMethod=Integration: Forward Euler  ExternalReset=level  LimitType=Anti-windup  B=2/F  A=-inf  Ts=Ts
  Periodic Difference (Discrete or Continuous) : eeGeneralMeasurement/Periodic Difference (Discrete or Continuous)  LabelModeActiveChoice=Continuous  F=F  Ts=Ts
      link override Continuous/Transport Delay: BufferSize=2^nextpow2(samplesPerPeriod*averageCycles+1024)
  Product : Product
  Real-Imag to Complex : RealImagToComplex
  SinCos : Subsystem
  Switch : Switch  Criteria=u2 > Threshold  Threshold=1/F  SaturateOnIntegerOverflow=off  InputSameDT=off
  RMS : Outport  VectorParamsAs1DForOutWhenUnconnected=off
  wires:
  Switch/1 -> RMS/1
  Gain2/1 -> Switch/1
  Constant2/1 -> Data Type Conversion Inherited2/2
  Constant3/1 -> Data Type Conversion Inherited1/2
  Constant4/1 -> Integrator (Discrete or Continuous)1/2
  Data Type Conversion Inherited3/1 -> Switch/3
  Constant5/1 -> Data Type Conversion Inherited3/2
  Data Type Conversion Inherited2/1 -> Integrator (Discrete or Continuous)1/1
  Data Type Conversion Inherited1/1 -> Integrator (Discrete or Continuous)1/3
  Integrator (Discrete or Continuous)1/1 -> Switch/2
  Constant1/1 -> Data Type Conversion Inherited/2
  Data Type Conversion Inherited/1 -> Integrator (Discrete or Continuous)/3
  Integrator (Discrete or Continuous)/1 -> Periodic Difference (Discrete or Continuous)/1
  Constant/1 -> Integrator (Discrete or Continuous)/2
  Demux/2 -> Real-Imag to Complex/2
  u/1 -> SinCos/1(u), Data Type Conversion Inherited/1, Data Type Conversion Inherited2/1, Data Type Conversion Inherited1/1, Data Type Conversion Inherited3/1, Product/1
  Periodic Difference (Discrete or Continuous)/1 -> Gain1/1
  Real-Imag to Complex/1 -> Complex to Magnitude-Angle/1
  Demux/1 -> Real-Imag to Complex/1
  SinCos/1(SinCos) -> Product/2
  Gain1/1 -> Demux/1
  Product/1 -> Integrator (Discrete or Continuous)/1
  Complex to Magnitude-Angle/1 -> Gain2/1

== system DWPT_250k_60V_1200W/RMS8/RMS Measurement/Total RMS ==
  u : Inport
  Constant{,1,3..4} (4 alike) : Constant  Value=0
  Constant2 : Constant
  Constant5 : Constant  Value=InitialRMS(1)
  Data Type Conversion Inherited{,1..3} (4 alike) : sl_signal_attributes/Data Type Conversion Inherited  ConvertRealWorld=Real World Value  DoSatur=off
  Gain : Gain  Gain=F
  Integrator (Discrete or Continuous) : eeGeneralControl/Integrator (Discrete or Continuous)  LabelModeActiveChoice=Continuous  IntegratorMethod=Integration: Forward Euler  ExternalReset=level  LimitType=Anti-windup  B=inf  A=-inf  Ts=Ts
  Integrator (Discrete or Continuous)1 : eeGeneralControl/Integrator (Discrete or Continuous)  LabelModeActiveChoice=Continuous  IntegratorMethod=Integration: Forward Euler  ExternalReset=level  LimitType=Anti-windup  B=2/F  A=-inf  Ts=Ts
  Math Function : Math  Operator=square  SignedPower=on
  Nonnegative mean square : Saturate  UpperLimit=inf  LowerLimit=0
  Periodic Difference (Discrete or Continuous) : eeGeneralMeasurement/Periodic Difference (Discrete or Continuous)  LabelModeActiveChoice=Continuous  F=F  Ts=Ts
      link override Continuous/Transport Delay: BufferSize=2^nextpow2(samplesPerPeriod*averageCycles+1024)
  Sqrt : Sqrt
  Switch : Switch  Criteria=u2 > Threshold  Threshold=1/F  SaturateOnIntegerOverflow=off  InputSameDT=off
  RMS : Outport  VectorParamsAs1DForOutWhenUnconnected=off
  wires:
  Sqrt/1 -> Switch/1
  Switch/1 -> RMS/1
  Constant2/1 -> Data Type Conversion Inherited2/2
  Constant3/1 -> Data Type Conversion Inherited1/2
  Constant4/1 -> Integrator (Discrete or Continuous)1/2
  Data Type Conversion Inherited3/1 -> Switch/3
  Constant5/1 -> Data Type Conversion Inherited3/2
  Data Type Conversion Inherited2/1 -> Integrator (Discrete or Continuous)1/1
  Data Type Conversion Inherited1/1 -> Integrator (Discrete or Continuous)1/3
  Integrator (Discrete or Continuous)1/1 -> Switch/2
  Constant1/1 -> Data Type Conversion Inherited/2
  Data Type Conversion Inherited/1 -> Integrator (Discrete or Continuous)/3
  Periodic Difference (Discrete or Continuous)/1 -> Gain/1
  Integrator (Discrete or Continuous)/1 -> Periodic Difference (Discrete or Continuous)/1
  u/1 -> Math Function/1, Data Type Conversion Inherited2/1, Data Type Conversion Inherited3/1, Data Type Conversion Inherited1/1
  Math Function/1 -> Integrator (Discrete or Continuous)/1, Data Type Conversion Inherited/1
  Constant/1 -> Integrator (Discrete or Continuous)/2
  Gain/1 -> Nonnegative mean square/1
  Nonnegative mean square/1 -> Sqrt/1

== system DWPT_250k_60V_1200W/RMS1/RMS Measurement/Harmonic RMS/SinCos ==
  u : Inport
  Data Type Conversion Inherited : sl_signal_attributes/Data Type Conversion Inherited  ConvertRealWorld=Real World Value  DoSatur=off
  Integrator with Wrapped State (Discrete or Continuous) : eeGeneralControl/Integrator with Wrapped State (Discrete or Continuous)  LabelModeActiveChoice=Continuous  WrappedStateUpperValue=2*pi  WrappedStateLowerValue=0  x0=0  Ts=Ts
  Mux : Mux  Inputs=2
  Radial frequencies : Constant  Value=2*pi*F*K
  sincos : Trigonometry  Operator=sincos
  SinCos : Outport  VectorParamsAs1DForOutWhenUnconnected=off
  wires:
  u/1 -> Data Type Conversion Inherited/1
  Radial frequencies/1 -> Data Type Conversion Inherited/2
  Data Type Conversion Inherited/1 -> Integrator with Wrapped State (Discrete or Continuous)/1
  Integrator with Wrapped State (Discrete or Continuous)/1 -> sincos/1
  Mux/1 -> SinCos/1
  sincos/1 -> Mux/1
  sincos/2 -> Mux/2

== system DWPT_250k_60V_1200W/RMS10/RMS Measurement/Harmonic RMS/SinCos ==
  u : Inport
  Data Type Conversion Inherited : sl_signal_attributes/Data Type Conversion Inherited  ConvertRealWorld=Real World Value  DoSatur=off
  Integrator with Wrapped State (Discrete or Continuous) : eeGeneralControl/Integrator with Wrapped State (Discrete or Continuous)  LabelModeActiveChoice=Continuous  WrappedStateUpperValue=2*pi  WrappedStateLowerValue=0  x0=0  Ts=Ts
  Mux : Mux  Inputs=2
  Radial frequencies : Constant  Value=2*pi*F*K
  sincos : Trigonometry  Operator=sincos
  SinCos : Outport  VectorParamsAs1DForOutWhenUnconnected=off
  wires:
  u/1 -> Data Type Conversion Inherited/1
  Radial frequencies/1 -> Data Type Conversion Inherited/2
  Data Type Conversion Inherited/1 -> Integrator with Wrapped State (Discrete or Continuous)/1
  Integrator with Wrapped State (Discrete or Continuous)/1 -> sincos/1
  Mux/1 -> SinCos/1
  sincos/1 -> Mux/1
  sincos/2 -> Mux/2

== system DWPT_250k_60V_1200W/RMS2/RMS Measurement/Harmonic RMS/SinCos ==
  u : Inport
  Data Type Conversion Inherited : sl_signal_attributes/Data Type Conversion Inherited  ConvertRealWorld=Real World Value  DoSatur=off
  Integrator with Wrapped State (Discrete or Continuous) : eeGeneralControl/Integrator with Wrapped State (Discrete or Continuous)  LabelModeActiveChoice=Continuous  WrappedStateUpperValue=2*pi  WrappedStateLowerValue=0  x0=0  Ts=Ts
  Mux : Mux  Inputs=2
  Radial frequencies : Constant  Value=2*pi*F*K
  sincos : Trigonometry  Operator=sincos
  SinCos : Outport  VectorParamsAs1DForOutWhenUnconnected=off
  wires:
  u/1 -> Data Type Conversion Inherited/1
  Radial frequencies/1 -> Data Type Conversion Inherited/2
  Data Type Conversion Inherited/1 -> Integrator with Wrapped State (Discrete or Continuous)/1
  Integrator with Wrapped State (Discrete or Continuous)/1 -> sincos/1
  Mux/1 -> SinCos/1
  sincos/1 -> Mux/1
  sincos/2 -> Mux/2

== system DWPT_250k_60V_1200W/RMS3/RMS Measurement/Harmonic RMS/SinCos ==
  u : Inport
  Data Type Conversion Inherited : sl_signal_attributes/Data Type Conversion Inherited  ConvertRealWorld=Real World Value  DoSatur=off
  Integrator with Wrapped State (Discrete or Continuous) : eeGeneralControl/Integrator with Wrapped State (Discrete or Continuous)  LabelModeActiveChoice=Continuous  WrappedStateUpperValue=2*pi  WrappedStateLowerValue=0  x0=0  Ts=Ts
  Mux : Mux  Inputs=2
  Radial frequencies : Constant  Value=2*pi*F*K
  sincos : Trigonometry  Operator=sincos
  SinCos : Outport  VectorParamsAs1DForOutWhenUnconnected=off
  wires:
  u/1 -> Data Type Conversion Inherited/1
  Radial frequencies/1 -> Data Type Conversion Inherited/2
  Data Type Conversion Inherited/1 -> Integrator with Wrapped State (Discrete or Continuous)/1
  Integrator with Wrapped State (Discrete or Continuous)/1 -> sincos/1
  Mux/1 -> SinCos/1
  sincos/1 -> Mux/1
  sincos/2 -> Mux/2

== system DWPT_250k_60V_1200W/RMS4/RMS Measurement/Harmonic RMS/SinCos ==
  u : Inport
  Data Type Conversion Inherited : sl_signal_attributes/Data Type Conversion Inherited  ConvertRealWorld=Real World Value  DoSatur=off
  Integrator with Wrapped State (Discrete or Continuous) : eeGeneralControl/Integrator with Wrapped State (Discrete or Continuous)  LabelModeActiveChoice=Continuous  WrappedStateUpperValue=2*pi  WrappedStateLowerValue=0  x0=0  Ts=Ts
  Mux : Mux  Inputs=2
  Radial frequencies : Constant  Value=2*pi*F*K
  sincos : Trigonometry  Operator=sincos
  SinCos : Outport  VectorParamsAs1DForOutWhenUnconnected=off
  wires:
  u/1 -> Data Type Conversion Inherited/1
  Radial frequencies/1 -> Data Type Conversion Inherited/2
  Data Type Conversion Inherited/1 -> Integrator with Wrapped State (Discrete or Continuous)/1
  Integrator with Wrapped State (Discrete or Continuous)/1 -> sincos/1
  Mux/1 -> SinCos/1
  sincos/1 -> Mux/1
  sincos/2 -> Mux/2

== system DWPT_250k_60V_1200W/RMS6/RMS Measurement/Harmonic RMS/SinCos ==
  u : Inport
  Data Type Conversion Inherited : sl_signal_attributes/Data Type Conversion Inherited  ConvertRealWorld=Real World Value  DoSatur=off
  Integrator with Wrapped State (Discrete or Continuous) : eeGeneralControl/Integrator with Wrapped State (Discrete or Continuous)  LabelModeActiveChoice=Continuous  WrappedStateUpperValue=2*pi  WrappedStateLowerValue=0  x0=0  Ts=Ts
  Mux : Mux  Inputs=2
  Radial frequencies : Constant  Value=2*pi*F*K
  sincos : Trigonometry  Operator=sincos
  SinCos : Outport  VectorParamsAs1DForOutWhenUnconnected=off
  wires:
  u/1 -> Data Type Conversion Inherited/1
  Radial frequencies/1 -> Data Type Conversion Inherited/2
  Data Type Conversion Inherited/1 -> Integrator with Wrapped State (Discrete or Continuous)/1
  Integrator with Wrapped State (Discrete or Continuous)/1 -> sincos/1
  Mux/1 -> SinCos/1
  sincos/1 -> Mux/1
  sincos/2 -> Mux/2

== system DWPT_250k_60V_1200W/RMS8/RMS Measurement/Harmonic RMS/SinCos ==
  u : Inport
  Data Type Conversion Inherited : sl_signal_attributes/Data Type Conversion Inherited  ConvertRealWorld=Real World Value  DoSatur=off
  Integrator with Wrapped State (Discrete or Continuous) : eeGeneralControl/Integrator with Wrapped State (Discrete or Continuous)  LabelModeActiveChoice=Continuous  WrappedStateUpperValue=2*pi  WrappedStateLowerValue=0  x0=0  Ts=Ts
  Mux : Mux  Inputs=2
  Radial frequencies : Constant  Value=2*pi*F*K
  sincos : Trigonometry  Operator=sincos
  SinCos : Outport  VectorParamsAs1DForOutWhenUnconnected=off
  wires:
  u/1 -> Data Type Conversion Inherited/1
  Radial frequencies/1 -> Data Type Conversion Inherited/2
  Data Type Conversion Inherited/1 -> Integrator with Wrapped State (Discrete or Continuous)/1
  Integrator with Wrapped State (Discrete or Continuous)/1 -> sincos/1
  Mux/1 -> SinCos/1
  sincos/1 -> Mux/1
  sincos/2 -> Mux/2

== matlab function DWPT_250k_60V_1200W/Synchronous rectifier control ==
  data: current input; positive output; negative output; Ts parameter; srDeadTime parameter; srThreshold parameter; srEnabled parameter
function [positive,negative] = sr_control(current, Ts, srDeadTime, srThreshold, srEnabled)
%#codegen
% Parameters: Ts, srDeadTime, srThreshold, srEnabled.
% Input is delayed one sample to avoid a physical-network algebraic loop.
% Turn off near zero current; require a stable polarity before turning on.
persistent previous stable
if isempty(previous)
    previous=0; stable=0;
end
polarity=0;
if current>srThreshold
    polarity=1;
elseif current<-srThreshold
    polarity=-1;
end
if polarity~=previous || polarity==0
    stable=0;
else
    stable=min(stable+1,ceil(srDeadTime/Ts)+1);
end
previous=polarity;
ready=stable>=ceil(srDeadTime/Ts) && srEnabled>0;
positive=double(ready && polarity==1);
negative=double(ready && polarity==-1);
end

== matlab function DWPT_250k_60V_1200W/Inverter control ==
  data: t input; g1 output; vout input; g2 output; g3 output; g4 output; modulation output; reference output; f parameter; Ts parameter; Vtarget parameter; Vavailable parameter; softStart parameter; deadTime parameter; Kp parameter; Ki parameter; closedLoop parameter
function [g1,g2,g3,g4,modulation,reference] = pwm_control(t,vout, f, Ts, Vtarget, Vavailable, softStart, deadTime, Kp, Ki, closedLoop)
%#codegen
% Parameters: f, Ts, Vtarget, Vavailable, softStart, deadTime, Kp, Ki, closedLoop.
% Update phase only at period boundaries to avoid mid-cycle gate glitches.
persistent integral command last1 last2 last3 last4 off1 off2 off3 off4
if isempty(integral)
    integral=0; command=0;
    last1=0;last2=0;last3=0;last4=0;
    off1=0;off2=0;off3=0;off4=0;
end
N=round(1/(f*Ts));
tick=mod(round(t/Ts),N);
reference=Vtarget*min(t/softStart,1);
if tick==0
    error=reference-vout;
    feedforward=reference/Vavailable;
    u=feedforward+closedLoop*(Kp*error+integral);
    command=min(max(u,0),1);
    if closedLoop>0 && ((u>0 && u<1) || (u>=1 && error<0) || (u<=0 && error>0))
        integral=min(max(integral+Ki*error/f,-1),1);
    end
end
shift=round(N*asin(command)/pi);
dead=round(deadTime/Ts);
phaseB=mod(tick-shift,N);
% Enforce interlock even when the phase command moves a carrier edge.
off1=min((off1+1)*(last1==0),dead+1);
off2=min((off2+1)*(last2==0),dead+1);
off3=min((off3+1)*(last3==0),dead+1);
off4=min((off4+1)*(last4==0),dead+1);
g1=double(tick>=dead && tick<N/2 && off2>=dead);
g2=double(tick>=N/2+dead && tick<N && off1>=dead);
g3=double(phaseB>=dead && phaseB<N/2 && off4>=dead);
g4=double(phaseB>=N/2+dead && phaseB<N && off3>=dead);
last1=g1;last2=g2;last3=g3;last4=g4;
modulation=command;
end
